simulink model "CellCal"  (R2024a)
settings: Solver=FixedStepDiscrete  StartTime=0.0  StopTime=10  FixedStep=0.01  RelTol=1e-3
PreLoadFcn:
  | if exist('CellCal_types', 'file') == 2, CellCal_types(); end
model workspace (MAT data in the model file):
  GainMax_code = Simulink.Parameter
  GainMax_code.Value = 11000
  GainMax_code.Complexity = 'real'
  GainMax_code.Dimensions = [1 1]
  GainMax_code.DataType = 'uint16'
  GainMin_code = Simulink.Parameter
  GainMin_code.Value = 9000
  GainMin_code.Complexity = 'real'
  GainMin_code.Dimensions = [1 1]
  GainMin_code.DataType = 'uint16'
  OffsetLimit_code = Simulink.Parameter
  OffsetLimit_code.Value = 2000
  OffsetLimit_code.Complexity = 'real'
  OffsetLimit_code.Dimensions = [1 1]
  OffsetLimit_code.DataType = 'uint16'
values from neighbouring files (symbols this model uses):
  GainMax_code = 11000    [CellCal_data.m]
  GainMin_code = 9000    [CellCal_data.m]
  OffsetLimit_code = 2000    [CellCal_data.m]
undefined symbols (not defined in the file or in its folder): QLF_NOT_AVAILABLE, QLF_OK
Description:
  | Kalibrierung der Zellkanaele: Werte per Diagnose uebernehmen (nur bei Ausgang aus), im NvM halten, an CellChannels geben
settings Model: ParameterArgumentNames=OffsetLimit_code,GainMin_code,GainMax_code  Creator=danie  LastModifiedBy=danie
settings OptimizationCC: DefaultParameterBehavior=Inlined  EnhancedBackFolding=on  PassReuseOutputArgsAs=Individual arguments  ZeroExternalMemoryAtStartup=off  ZeroInternalMemoryAtStartup=off  OptimizeBlockOrder=speed  DifferentSizesBufferReuse=on  OptimizationCustomize=off  EfficientTunableParamExpr=on
settings DebuggingCC: ParameterTunabilityLossMsg=error
settings HardwareCC: ProdBitPerPointer=32  ProdBitPerSizeT=32  ProdBitPerPtrDiffT=32  ProdLargestAtomicInteger=Long  ProdLargestAtomicFloat=Double  ProdWordSize=32  ProdLongLongMode=on  ProdHWDeviceType=ARM Compatible->ARM Cortex-M
settings SFSimCC: MATLABDynamicMemAlloc=off
settings RTWCC: Description=AUTOSAR  SystemTargetFile=autosar.tlc  GenCodeOnly=on  GenerateMakefile=off  TemplateMakefile=ert_default_tmf  DataTypeReplacement=CDataTypesFixedWidth
settings CodeAppCC: ForceParamTrailComments=on  IgnoreCustomStorageClasses=off  MaxIdLength=63  OperatorAnnotations=on  SimulinkDataObjDesc=on  SFDataObjDesc=on  InsertBlockDesc=on
settings STFCustomTargetCC: MultiwordLength=256  ParMdlRefBuildCompliant=on  CompOptLevelCompliant=on  IncludeMdlTerminateFcn=off  CombineOutputUpdateFcns=on  SuppressErrorStatus=on  ERTCustomFileBanners=on  SupportNonFinite=off  SupportComplex=off  SupportContinuousTime=off  SupportNonInlinedSFcns=off  RemoveResetFunc=on  MATLABClassNameForMDSCustomization=Simulink.SoftwareTarget.ERTCustomization  AutosarCompliant=on  GRTInterface=off  LookupTableObjectStructAxisOrder=2,1,3,4,...  LUTObjectStructOrderEvenSpacing=Size,Table,Breakpoints  SystemTargetFile=autosar.tlc
settings ERTTargetCC: TargetLangStandard=C99 (ISO)  ConcurrentExecutionCompliant=off  IncludeMdlTerminateFcn=off  SuppressErrorStatus=on  SupportNonFinite=off  SupportComplex=off  ModelStepFunctionPrototypeControlCompliant=off  CPPClassGenCompliant=off  AutosarCompliant=on  LookupTableObjectStructAxisOrder=2,1,3,4,...  LUTObjectStructOrderEvenSpacing=Size,Table,Breakpoints  InlinedParameterPlacement=NonHierarchical  ERTCustomFileTemplate=example_file_process.tlc  BooleanTrueId=TRUE  BooleanFalseId=FALSE

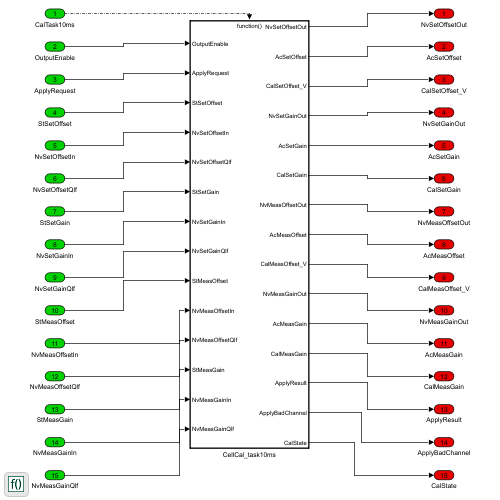
[thumbnail: Simulink's stored preview of the top-level diagram]
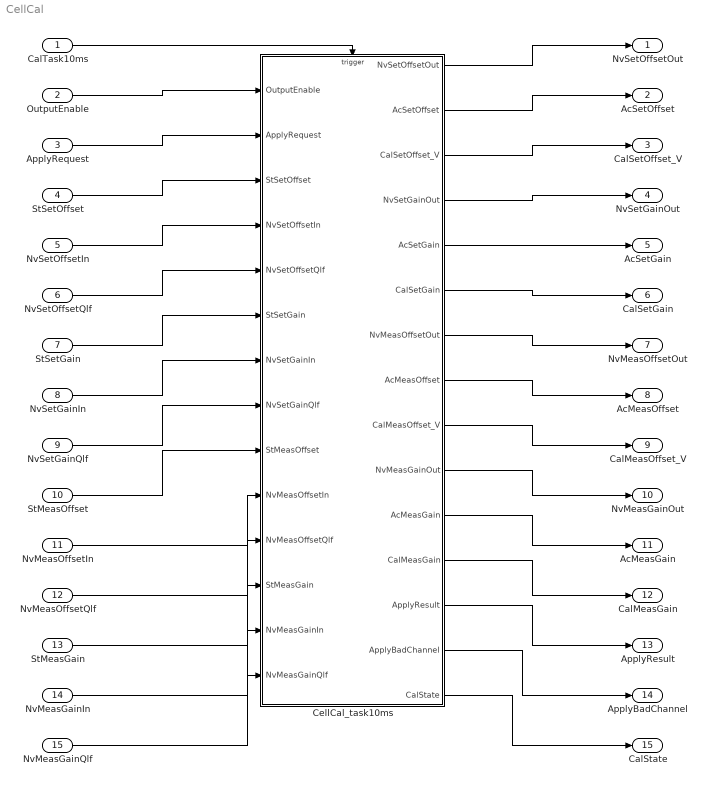
== system CellCal ==
  CalTask10ms : Inport  SampleTime=0.01  OutputFunctionCall=on
  OutputEnable : Inport  Port=2  OutDataTypeStr=boolean  PortDimensions=1
  ApplyRequest : Inport  Port=3  OutDataTypeStr=uint8  PortDimensions=1
  StSetOffset : Inport  Port=4  OutDataTypeStr=int16  PortDimensions=CellCount
  NvSetOffsetIn : Inport  Port=5  OutDataTypeStr=int16  PortDimensions=CellCount
  NvSetOffsetQlf : Inport  Port=6  OutDataTypeStr=uint8  PortDimensions=1
  StSetGain : Inport  Port=7  OutDataTypeStr=uint16  PortDimensions=CellCount
  NvSetGainIn : Inport  Port=8  OutDataTypeStr=uint16  PortDimensions=CellCount
  NvSetGainQlf : Inport  Port=9  OutDataTypeStr=uint8  PortDimensions=1
  StMeasOffset : Inport  Port=10  OutDataTypeStr=int16  PortDimensions=CellCount
  NvMeasOffsetIn : Inport  Port=11  OutDataTypeStr=int16  PortDimensions=CellCount
  NvMeasOffsetQlf : Inport  Port=12  OutDataTypeStr=uint8  PortDimensions=1
  StMeasGain : Inport  Port=13  OutDataTypeStr=uint16  PortDimensions=CellCount
  NvMeasGainIn : Inport  Port=14  OutDataTypeStr=uint16  PortDimensions=CellCount
  NvMeasGainQlf : Inport  Port=15  OutDataTypeStr=uint8  PortDimensions=1
  CellCal_task10ms : Subsystem  TreatAsAtomicUnit=on
  NvSetOffsetOut : Outport  OutDataTypeStr=int16  PortDimensions=CellCount
  AcSetOffset : Outport  Port=2  OutDataTypeStr=int16  PortDimensions=CellCount
  CalSetOffset_V : Outport  Port=3  OutDataTypeStr=single  PortDimensions=CellCount
  NvSetGainOut : Outport  Port=4  OutDataTypeStr=uint16  PortDimensions=CellCount
  AcSetGain : Outport  Port=5  OutDataTypeStr=uint16  PortDimensions=CellCount
  CalSetGain : Outport  Port=6  OutDataTypeStr=single  PortDimensions=CellCount
  NvMeasOffsetOut : Outport  Port=7  OutDataTypeStr=int16  PortDimensions=CellCount
  AcMeasOffset : Outport  Port=8  OutDataTypeStr=int16  PortDimensions=CellCount
  CalMeasOffset_V : Outport  Port=9  OutDataTypeStr=single  PortDimensions=CellCount
  NvMeasGainOut : Outport  Port=10  OutDataTypeStr=uint16  PortDimensions=CellCount
  AcMeasGain : Outport  Port=11  OutDataTypeStr=uint16  PortDimensions=CellCount
  CalMeasGain : Outport  Port=12  OutDataTypeStr=single  PortDimensions=CellCount
  ApplyResult : Outport  Port=13  OutDataTypeStr=uint8  PortDimensions=1
  ApplyBadChannel : Outport  Port=14  OutDataTypeStr=uint8  PortDimensions=1
  CalState : Outport  Port=15  OutDataTypeStr=uint8  PortDimensions=1
  wires:
  CalTask10ms/1 -> CellCal_task10ms/Trigger
  OutputEnable/1 -> CellCal_task10ms/1(OutputEnable)
  ApplyRequest/1 -> CellCal_task10ms/2(ApplyRequest)
  StSetOffset/1 -> CellCal_task10ms/3(StSetOffset)
  NvSetOffsetIn/1 -> CellCal_task10ms/4(NvSetOffsetIn)
  NvSetOffsetQlf/1 -> CellCal_task10ms/5(NvSetOffsetQlf)
  StSetGain/1 -> CellCal_task10ms/6(StSetGain)
  NvSetGainIn/1 -> CellCal_task10ms/7(NvSetGainIn)
  NvSetGainQlf/1 -> CellCal_task10ms/8(NvSetGainQlf)
  StMeasOffset/1 -> CellCal_task10ms/9(StMeasOffset)
  NvMeasOffsetIn/1 -> CellCal_task10ms/10(NvMeasOffsetIn)
  NvMeasOffsetQlf/1 -> CellCal_task10ms/11(NvMeasOffsetQlf)
  StMeasGain/1 -> CellCal_task10ms/12(StMeasGain)
  NvMeasGainIn/1 -> CellCal_task10ms/13(NvMeasGainIn)
  NvMeasGainQlf/1 -> CellCal_task10ms/14(NvMeasGainQlf)
  CellCal_task10ms/1(NvSetOffsetOut) -> NvSetOffsetOut/1
  CellCal_task10ms/2(AcSetOffset) -> AcSetOffset/1
  CellCal_task10ms/3(CalSetOffset_V) -> CalSetOffset_V/1
  CellCal_task10ms/4(NvSetGainOut) -> NvSetGainOut/1
  CellCal_task10ms/5(AcSetGain) -> AcSetGain/1
  CellCal_task10ms/6(CalSetGain) -> CalSetGain/1
  CellCal_task10ms/7(NvMeasOffsetOut) -> NvMeasOffsetOut/1
  CellCal_task10ms/8(AcMeasOffset) -> AcMeasOffset/1
  CellCal_task10ms/9(CalMeasOffset_V) -> CalMeasOffset_V/1
  CellCal_task10ms/10(NvMeasGainOut) -> NvMeasGainOut/1
  CellCal_task10ms/11(AcMeasGain) -> AcMeasGain/1
  CellCal_task10ms/12(CalMeasGain) -> CalMeasGain/1
  CellCal_task10ms/13(ApplyResult) -> ApplyResult/1
  CellCal_task10ms/14(ApplyBadChannel) -> ApplyBadChannel/1
  CellCal_task10ms/15(CalState) -> CalState/1

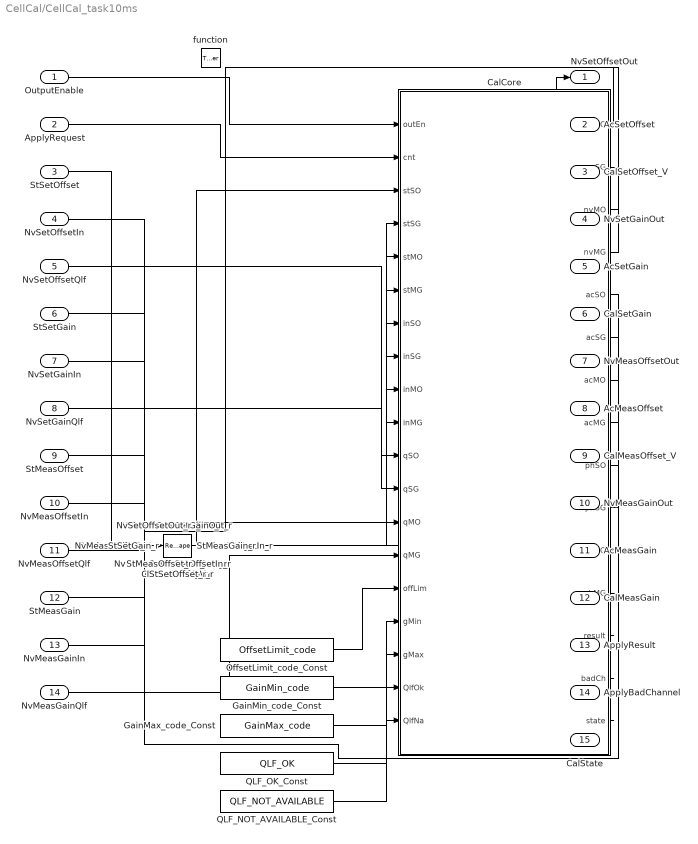
== system CellCal/CellCal_task10ms ==
  OutputEnable : Inport
  ApplyRequest : Inport  Port=2
  StSetOffset : Inport  Port=3
  NvSetOffsetIn : Inport  Port=4
  NvSetOffsetQlf : Inport  Port=5
  StSetGain : Inport  Port=6
  NvSetGainIn : Inport  Port=7
  NvSetGainQlf : Inport  Port=8
  StMeasOffset : Inport  Port=9
  NvMeasOffsetIn : Inport  Port=10
  NvMeasOffsetQlf : Inport  Port=11
  StMeasGain : Inport  Port=12
  NvMeasGainIn : Inport  Port=13
  NvMeasGainQlf : Inport  Port=14
  function : TriggerPort  TriggerType=function-call  VariantControl=(inherit)  SampleTimeType=periodic  SampleTime=0.01
  AcMeasGain_r : Reshape
  AcMeasOffset_r : Reshape
  AcSetGain_r : Reshape
  AcSetOffset_r : Reshape
  CalCore : MATLAB Function  TreatAsAtomicUnit=on
  CalMeasGain_r : Reshape
  CalMeasOffset_V_r : Reshape
  CalSetGain_r : Reshape
  CalSetOffset_V_r : Reshape
  GainMax_code_Const : Constant  Value=GainMax_code  OutDataTypeStr=uint16
  GainMin_code_Const : Constant  Value=GainMin_code  OutDataTypeStr=uint16
  NvMeasGainIn_r : Reshape  OutputDimensionality=Customize  OutputDimensions=[14 1]
  NvMeasGainOut_r : Reshape
  NvMeasOffsetIn_r : Reshape  OutputDimensionality=Customize  OutputDimensions=[14 1]
  NvMeasOffsetOut_r : Reshape
  NvSetGainIn_r : Reshape  OutputDimensionality=Customize  OutputDimensions=[14 1]
  NvSetGainOut_r : Reshape
  NvSetOffsetIn_r : Reshape  OutputDimensionality=Customize  OutputDimensions=[14 1]
  NvSetOffsetOut_r : Reshape
  OffsetLimit_code_Const : Constant  Value=OffsetLimit_code  OutDataTypeStr=uint16
  QLF_NOT_AVAILABLE_Const : Constant  Value=QLF_NOT_AVAILABLE  OutDataTypeStr=uint8
  QLF_OK_Const : Constant  Value=QLF_OK  OutDataTypeStr=uint8
  StMeasGain_r : Reshape  OutputDimensionality=Customize  OutputDimensions=[14 1]
  StMeasOffset_r : Reshape  OutputDimensionality=Customize  OutputDimensions=[14 1]
  StSetGain_r : Reshape  OutputDimensionality=Customize  OutputDimensions=[14 1]
  StSetOffset_r : Reshape  OutputDimensionality=Customize  OutputDimensions=[14 1]
  NvSetOffsetOut : Outport
  AcSetOffset : Outport  Port=2
  CalSetOffset_V : Outport  Port=3
  NvSetGainOut : Outport  Port=4
  AcSetGain : Outport  Port=5
  CalSetGain : Outport  Port=6
  NvMeasOffsetOut : Outport  Port=7
  AcMeasOffset : Outport  Port=8
  CalMeasOffset_V : Outport  Port=9
  NvMeasGainOut : Outport  Port=10
  AcMeasGain : Outport  Port=11
  CalMeasGain : Outport  Port=12
  ApplyResult : Outport  Port=13
  ApplyBadChannel : Outport  Port=14
  CalState : Outport  Port=15
  wires:
  StSetOffset/1 -> StSetOffset_r/1
  StSetGain/1 -> StSetGain_r/1
  StMeasOffset/1 -> StMeasOffset_r/1
  StMeasGain/1 -> StMeasGain_r/1
  NvSetOffsetIn/1 -> NvSetOffsetIn_r/1
  NvSetGainIn/1 -> NvSetGainIn_r/1
  NvMeasOffsetIn/1 -> NvMeasOffsetIn_r/1
  NvMeasGainIn/1 -> NvMeasGainIn_r/1
  NvSetOffsetOut_r/1 -> NvSetOffsetOut/1
  NvSetGainOut_r/1 -> NvSetGainOut/1
  NvMeasOffsetOut_r/1 -> NvMeasOffsetOut/1
  NvMeasGainOut_r/1 -> NvMeasGainOut/1
  AcSetOffset_r/1 -> AcSetOffset/1
  AcSetGain_r/1 -> AcSetGain/1
  AcMeasOffset_r/1 -> AcMeasOffset/1
  AcMeasGain_r/1 -> AcMeasGain/1
  CalSetOffset_V_r/1 -> CalSetOffset_V/1
  CalSetGain_r/1 -> CalSetGain/1
  CalMeasOffset_V_r/1 -> CalMeasOffset_V/1
  CalMeasGain_r/1 -> CalMeasGain/1
  OutputEnable/1 -> CalCore/1(outEn)
  ApplyRequest/1 -> CalCore/2(cnt)
  StSetOffset_r/1 -> CalCore/3(stSO)
  StSetGain_r/1 -> CalCore/4(stSG)
  StMeasOffset_r/1 -> CalCore/5(stMO)
  StMeasGain_r/1 -> CalCore/6(stMG)
  NvSetOffsetIn_r/1 -> CalCore/7(inSO)
  NvSetGainIn_r/1 -> CalCore/8(inSG)
  NvMeasOffsetIn_r/1 -> CalCore/9(inMO)
  NvMeasGainIn_r/1 -> CalCore/10(inMG)
  NvSetOffsetQlf/1 -> CalCore/11(qSO)
  NvSetGainQlf/1 -> CalCore/12(qSG)
  NvMeasOffsetQlf/1 -> CalCore/13(qMO)
  NvMeasGainQlf/1 -> CalCore/14(qMG)
  OffsetLimit_code_Const/1 -> CalCore/15(offLim)
  GainMin_code_Const/1 -> CalCore/16(gMin)
  GainMax_code_Const/1 -> CalCore/17(gMax)
  QLF_OK_Const/1 -> CalCore/18(QlfOk)
  QLF_NOT_AVAILABLE_Const/1 -> CalCore/19(QlfNa)
  CalCore/1(nvSO) -> NvSetOffsetOut_r/1
  CalCore/2(nvSG) -> NvSetGainOut_r/1
  CalCore/3(nvMO) -> NvMeasOffsetOut_r/1
  CalCore/4(nvMG) -> NvMeasGainOut_r/1
  CalCore/5(acSO) -> AcSetOffset_r/1
  CalCore/6(acSG) -> AcSetGain_r/1
  CalCore/7(acMO) -> AcMeasOffset_r/1
  CalCore/8(acMG) -> AcMeasGain_r/1
  CalCore/9(phSO) -> CalSetOffset_V_r/1
  CalCore/10(phSG) -> CalSetGain_r/1
  CalCore/11(phMO) -> CalMeasOffset_V_r/1
  CalCore/12(phMG) -> CalMeasGain_r/1
  CalCore/13(result) -> ApplyResult/1
  CalCore/14(badCh) -> ApplyBadChannel/1
  CalCore/15(state) -> CalState/1

== matlab function CellCal/CellCal_task10ms/CalCore ==
  data: outEn input; nvSO output; cnt input; stSO input; stSG input; stMO input; stMG input; inSO input; inSG input; inMO input; inMG input; qSO input; qSG input; qMO input; qMG input; offLim input; gMin input; gMax input; QlfOk input; QlfNa input; nvSG output; nvMO output; nvMG output; acSO output; acSG output; acMO output; acMG output; phSO output; phSG output; phMO output; phMG output; result output; badCh output; state output
function [nvSO, nvSG, nvMO, nvMG, acSO, acSG, acMO, acMG, phSO, phSG, phMO, phMG, result, badCh, state] = CalCore( ...
    outEn, cnt, stSO, stSG, stMO, stMG, inSO, inSG, inMO, inMG, qSO, qSG, qMO, qMG, offLim, gMin, gMax, QlfOk, QlfNa)
%CALCORE Calibration of 14 channels: stored values, staged values, takeover by request (see CalCell_create.m).
%#codegen
persistent aSO aSG aMO aMG last res bad st started
if isempty(started)
    started = true;
    [aSO, s1] = loadOffsets(inSO, qSO, offLim, QlfOk, QlfNa);
    [aSG, s2] = loadGains(inSG, qSG, gMin, gMax, QlfOk, QlfNa);
    [aMO, s3] = loadOffsets(inMO, qMO, offLim, QlfOk, QlfNa);
    [aMG, s4] = loadGains(inMG, qMG, gMin, gMax, QlfOk, QlfNa);
    st = max(max(s1, s2), max(s3, s4));
    last = cnt;
    res = uint8(3);
    bad = uint8(0);
end
if cnt ~= last
    last = cnt;
    res = uint8(3);
    bad = uint8(0);
    if outEn
        res = uint8(1);
    else
        req = false(14, 1);
        for k = 1:14
            written = (stSO(k) ~= int16(0)) || (stSG(k) ~= uint16(0)) || (stMO(k) ~= int16(0)) || (stMG(k) ~= uint16(0));
            differs = (stSO(k) ~= aSO(k)) || (stSG(k) ~= aSG(k)) || (stMO(k) ~= aMO(k)) || (stMG(k) ~= aMG(k));
            if written && differs
                req(k) = true;
                inRange = (abs(int32(stSO(k))) <= int32(offLim)) && (abs(int32(stMO(k))) <= int32(offLim)) && ...
                    (stSG(k) >= gMin) && (stSG(k) <= gMax) && (stMG(k) >= gMin) && (stMG(k) <= gMax);
                if ~inRange && bad == uint8(0)
                    bad = uint8(k);
                end
            end
        end
        if bad ~= uint8(0)
            res = uint8(2);
        elseif any(req)
            for k = 1:14
                if req(k)
                    aSO(k) = stSO(k);
                    aSG(k) = stSG(k);
                    aMO(k) = stMO(k);
                    aMG(k) = stMG(k);
                end
            end
            res = uint8(0);
            if st == uint8(0)
                st = uint8(1);
            end
        end
    end
end
nvSO = aSO; nvSG = aSG; nvMO = aMO; nvMG = aMG;
acSO = aSO; acSG = aSG; acMO = aMO; acMG = aMG;
phSO = single(aSO) * single(0.0001);
phSG = single(aSG) * single(0.0001);
phMO = single(aMO) * single(0.0001);
phMG = single(aMG) * single(0.0001);
result = res;
badCh = bad;
state = st;

function [v, s] = loadOffsets(inV, q, lim, QlfOk, QlfNa)
% stored offsets (a never written block delivers its default 0); the factory value 0 for a defective block or a value outside the limit
v = zeros(14, 1, 'int16');
s = uint8(0);
if (q == QlfOk) || (q == QlfNa)
    if q == QlfOk
        s = uint8(1);
    end
    for k = 1:14
        if abs(int32(inV(k))) <= int32(lim)
            v(k) = inV(k);
        else
            s = uint8(2);
        end
    end
elseif q ~= QlfNa
    s = uint8(2);
end

function [v, s] = loadGains(inV, q, lo, hi, QlfOk, QlfNa)
% stored gains (a never written block delivers its default 1.0000, code 10000, from the initial value of the port); the factory value
% 1.0000 for a defective block or a value outside the limits
v = uint16(10000) * ones(14, 1, 'uint16');
s = uint8(0);
if (q == QlfOk) || (q == QlfNa)
    if q == QlfOk
        s = uint8(1);
    end
    for k = 1:14
        if (inV(k) >= lo) && (inV(k) <= hi)
            v(k) = inV(k);
        else
            s = uint8(2);
        end
    end
elseif q ~= QlfNa
    s = uint8(2);
end
